simulink model "P642_VTS_Reference"  (R2026b)
settings: Solver=FixedStepDiscrete  StopTime=5  FixedStep=0.001
libraries: simulink_extras x4
settings Model: Creator=Medha Trust  LastModifiedBy=Medha Trust
settings DataIOCC: ExternalInput=input_data  LoadExternalInput=on

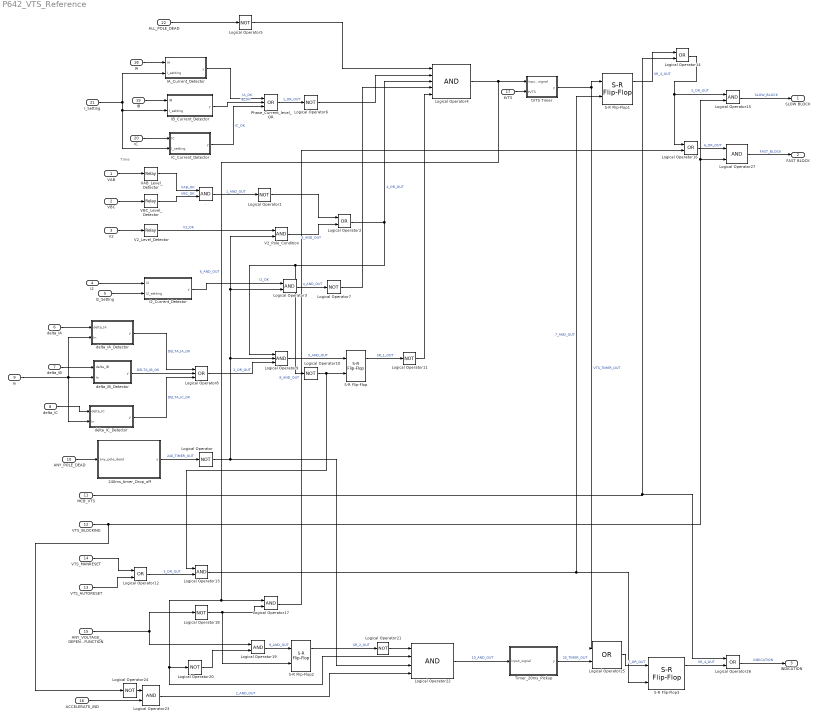
== system P642_VTS_Reference ==
  note: Time
  VAB : Inport
  VBC : Inport  Port=2
  V2 : Inport  Port=3  OutDataTypeStr=double
  I2 : Inport  Port=4
  I2_Setting : Inport  Port=5
  delta_IA : Inport  Port=6
  delta_IB : Inport  Port=7
  delta_IC : Inport  Port=8
  In : Inport  Port=9
  ANY_POLE_DEAD : Inport  Port=10
  MCB_VTS : Inport  Port=11  OutDataTypeStr=double
  VTS_BLOCKING : Inport  Port=12  OutDataTypeStr=double
  VTS_AUTORESET : Inport  Port=13  OutDataTypeStr=double
  VTS_MANRESET : Inport  Port=14  OutDataTypeStr=double
  ANY_VOLTAGE_DEPENDENT_FUNCTION : Inport  Port=15  OutDataTypeStr=double
  ACCELERATE_IND : Inport  Port=16  OutDataTypeStr=double
  tVTS : Inport  Port=17
  IA : Inport  Port=18
  IB : Inport  Port=19
  IC : Inport  Port=20
  I_Setting : Inport  Port=21
  ALL_POLE_DEAD : Inport  Port=22  OutDataTypeStr=double
  " ." : Logic  AllPortsSameDT=off  OutDataTypeStr=boolean
  240ms_timer_Drop_off : MATLAB Function  TreatAsAtomicUnit=on
  I2_Current_Detector : MATLAB Function  TreatAsAtomicUnit=on
  IA_Current_Detector : MATLAB Function  TreatAsAtomicUnit=on
  IB_Current_Detector : MATLAB Function  TreatAsAtomicUnit=on
  IC_Current_Detector : MATLAB Function  TreatAsAtomicUnit=on
  Logical Operator{,1,5..7,10..11,18,20..21,24} (11 alike) : Logic  Operator=NOT  AllPortsSameDT=off  OutDataTypeStr=boolean
  Logical Operator{2,12,14,16,25..26} (6 alike) : Logic  Operator=OR  AllPortsSameDT=off  OutDataTypeStr=boolean
  Logical Operator{3,13,15,17,19,23,27} (7 alike) : Logic  AllPortsSameDT=off  OutDataTypeStr=boolean
  Logical Operator22 : Logic  Inputs=4  AllPortsSameDT=off  OutDataTypeStr=boolean
  Logical Operator4 : Logic  Inputs=5  AllPortsSameDT=off  OutDataTypeStr=boolean
  Logical Operator8 : Logic  Operator=OR  Inputs=3  AllPortsSameDT=off  OutDataTypeStr=boolean
  Logical Operator9 : Logic  Inputs=3  AllPortsSameDT=off  OutDataTypeStr=boolean
  Phase_Current_level_OR : Logic  Operator=OR  Inputs=3  AllPortsSameDT=off  OutDataTypeStr=boolean
  S-R Flip-Flop{,1..3} (4 alike) : simulink_extras/Flip Flops/S-R Flip-Flop  initial_condition=0
  Timer_20ms_Pickup : MATLAB Function  TreatAsAtomicUnit=on
  V2_Level_Detector : Relay  OnSwitchValue=10  OffSwitchValue=9.5
  V2_Pole_Condition : Logic  AllPortsSameDT=off  OutDataTypeStr=boolean
  VAB_Level_Detector : Relay  OnSwitchValue=95  OffSwitchValue=70
  VBC_Level_Detector : Relay  OnSwitchValue=95  OffSwitchValue=70
  delta_IA_Detector : MATLAB Function  TreatAsAtomicUnit=on
  delta_IB_Detector : MATLAB Function  TreatAsAtomicUnit=on
  delta_IC_Detector : MATLAB Function  TreatAsAtomicUnit=on
  tVTS Timer : MATLAB Function  TreatAsAtomicUnit=on
  SLOW BLOCK : Outport
  FAST BLOCK : Outport  Port=2
  INDICATION : Outport  Port=3
  wires:
  VAB/1 -> VAB_Level_Detector/1
  VAB_Level_Detector/1 -> " ."/1  "VAB_OK"
  VBC/1 -> VBC_Level_Detector/1
  VBC_Level_Detector/1 -> " ."/2  "VBC_OK"
  V2/1 -> V2_Level_Detector/1
  V2_Level_Detector/1 -> V2_Pole_Condition/1  "V2_OK"
  I2/1 -> I2_Current_Detector/1(I2)
  I2_Setting/1 -> I2_Current_Detector/2(I2_setting)
  I2_Current_Detector/1(y) -> Logical Operator3/1  "I2_OK"
  delta_IA/1 -> delta_IA_Detector/1(delta_IA)
  In/1 -> delta_IC_Detector/2(In), delta_IB_Detector/2(In), delta_IA_Detector/2(In)
  delta_IB/1 -> delta_IB_Detector/1(delta_IB)
  delta_IC/1 -> delta_IC_Detector/1(delta_IC)
  Logical Operator/1 -> Logical Operator22/3, Logical Operator3/2, V2_Pole_Condition/2, Logical Operator9/2
  " ."/1 -> Logical Operator1/1  "1_AND_OUT"
  Logical Operator1/1 -> Logical Operator2/1
  V2_Pole_Condition/1 -> Logical Operator2/2  "3_AND_OUT"
  IB_Current_Detector/1(y) -> Phase_Current_level_OR/2  "IB_OK"
  IC/1 -> IC_Current_Detector/1(IC)
  IB/1 -> IB_Current_Detector/1(IB)
  I_Setting/1 -> IA_Current_Detector/2(I_setting), IC_Current_Detector/2(I_setting), IB_Current_Detector/2(I_setting)
  IA/1 -> IA_Current_Detector/1(IA)
  IC_Current_Detector/1(y) -> Phase_Current_level_OR/3  "IC_OK"
  IA_Current_Detector/1(y) -> Phase_Current_level_OR/1  "IA_OK"
  ALL_POLE_DEAD/1 -> Logical Operator5/1
  Logical Operator5/1 -> Logical Operator4/1
  Phase_Current_level_OR/1 -> Logical Operator6/1  "1_OR_OUT"
  Logical Operator6/1 -> Logical Operator4/2
  Logical Operator2/1 -> Logical Operator10/1, Logical Operator9/1, Logical Operator4/3  "4_OR_OUT"
  Logical Operator3/1 -> Logical Operator7/1  "4_AND_OUT"
  Logical Operator7/1 -> Logical Operator4/4
  delta_IA_Detector/1(y) -> Logical Operator8/1  "DELTA_IA_OK"
  delta_IB_Detector/1(y) -> Logical Operator8/2  "DELTA_IB_OK"
  delta_IC_Detector/1(y) -> Logical Operator8/3  "DELTA_IC_OK"
  Logical Operator8/1 -> Logical Operator9/3  "2_OR_OUT"
  Logical Operator9/1 -> S-R Flip-Flop/1  "5_AND_OUT"
  Logical Operator10/1 -> Logical Operator13/1, S-R Flip-Flop/2
  S-R Flip-Flop/1 -> Logical Operator11/1  "SR_1_OUT"
  Logical Operator11/1 -> Logical Operator4/5
  VTS_MANRESET/1 -> Logical Operator12/1
  VTS_AUTORESET/1 -> Logical Operator12/2
  Logical Operator12/1 -> Logical Operator13/2  "3_OR_OUT"
  tVTS/1 -> tVTS Timer/2(tVTS)
  Logical Operator4/1 -> tVTS Timer/1(input_signal), Logical Operator17/1, Logical Operator22/2, Logical Operator20/1  "6_AND_OUT"
  Logical Operator13/1 -> S-R Flip-Flop3/2, S-R Flip-Flop1/2  "7_AND_OUT"
  S-R Flip-Flop1/1 -> Logical Operator14/1  "SR_3_OUT"
  MCB_VTS/1 -> Logical Operator26/1, Logical Operator14/2
  Logical Operator14/1 -> Logical Operator15/1, Logical Operator16/1  "5_OR_OUT"
  VTS_BLOCKING/1 -> Logical Operator27/2, Logical Operator15/2, Logical Operator24/1
  ANY_VOLTAGE_DEPENDENT_FUNCTION/1 -> Logical Operator19/1, Logical Operator18/1
  Logical Operator18/1 -> S-R Flip-Flop2/2, Logical Operator17/2
  Logical Operator17/1 -> Logical Operator16/2  "8_AND_OUT"
  Logical Operator20/1 -> Logical Operator19/2
  Logical Operator19/1 -> S-R Flip-Flop2/1  "9_AND_OUT"
  S-R Flip-Flop2/1 -> Logical Operator21/1  "SR_2_OUT"
  Logical Operator21/1 -> Logical Operator22/1
  Logical Operator24/1 -> Logical Operator23/1
  ACCELERATE_IND/1 -> Logical Operator23/2
  Logical Operator23/1 -> Logical Operator22/4  "2_AND_OUT"
  ANY_POLE_DEAD/1 -> 240ms_timer_Drop_off/1(any_pole_dead)
  240ms_timer_Drop_off/1(y) -> Logical Operator/1  "240_TIMER_OUT"
  tVTS Timer/1(y) -> S-R Flip-Flop1/1, Logical Operator25/1  "VTS_TIMER_OUT"
  Logical Operator22/1 -> Timer_20ms_Pickup/1(input_signal)  "10_AND_OUT"
  Timer_20ms_Pickup/1(y) -> Logical Operator25/2  "20_TIMER_OUT"
  Logical Operator25/1 -> S-R Flip-Flop3/1  "7_OR_OUT"
  S-R Flip-Flop3/1 -> Logical Operator26/2  "SR_4_OUT"
  Logical Operator16/1 -> Logical Operator27/1  "6_OR_OUT"
  Logical Operator26/1 -> INDICATION/1  "INDICATION"
  Logical Operator27/1 -> FAST BLOCK/1  "FAST_BLOCK"
  Logical Operator15/1 -> SLOW BLOCK/1  "SLOW_BLOCK"

== matlab function P642_VTS_Reference/IA_Current_Detector ==
  data: IA input; y output; I_setting input
function y = fcn(IA, I_setting)
% P642 IA> current level detector
% Pickup  = 100% of I> setting
% Dropout = 95% of I> setting

persistent state

if isempty(state)
    state = 0;
end

pickup = I_setting;
dropout = 0.95 * I_setting;

if state == 0
    if abs(IA) >= pickup
        state = 1;
    end
else
    if abs(IA) < dropout
        state = 0;
    end
end

y = logical(state);

== matlab function P642_VTS_Reference/IC_Current_Detector ==
  data: IC input; y output; I_setting input
function y = fcn(IC, I_setting)

y=false; %Initializing input
% P642 IA> current level detector
% Pickup  = 100% of I> setting
% Dropout = 95% of I> setting

persistent state

if isempty(state)
    state = 0;
end

pickup = I_setting;
dropout = 0.95 * I_setting;

if state == 0
    if abs(IC) >= pickup
        state = 1;
    end
else
    if abs(IC) < dropout
        state = 0;
    end
end

y = logical(state);

== matlab function P642_VTS_Reference/I2_Current_Detector ==
  data: I2 input; y output boolean; I2_setting input
function y = fcn(I2, I2_setting)
% P642 I2> negative-sequence current detector
% Pickup  = 100% of I2> setting
% Dropout = 95% of I2> setting

persistent state

if isempty(state)
    state = 0;
end

pickup = I2_setting;
dropout = 0.95 * I2_setting;

if state == 0
    if abs(I2) >= pickup
        state = 1;
    end
else
    if abs(I2) < dropout
        state = 0;
    end
end

y = logical(state);

== matlab function P642_VTS_Reference/delta_IA_Detector ==
  data: delta_IA input; y output; In input
function y = fcn(delta_IA, In)
% P642 Delta IA> superimposed-current detector
% Threshold = 0.1 * In
% Operate decision must persist for 0.5 cycle
% Simulation step = 0.001 s
% Nominal frequency = 50 Hz
% Therefore 0.5 cycle = 0.01 s = 10 samples

persistent count state

if isempty(count)
    count = 0;
    state = 0;
end

threshold = 0.1 * In;
required_samples = 10;

if abs(delta_IA) >= threshold
    count = count + 1;
else
    count = 0;
    state = 0;
end

if count >= required_samples
    state = 1;
end

y = state;

== matlab function P642_VTS_Reference/delta_IB_Detector ==
  data: delta_IB input; y output; In input
function y = fcn(delta_IB, In)
% P642 Delta IA> superimposed-current detector
% Threshold = 0.1 * In
% Operate decision must persist for 0.5 cycle
% Simulation step = 0.001 s
% Nominal frequency = 50 Hz
% Therefore 0.5 cycle = 0.01 s = 10 samples

persistent count state

if isempty(count)
    count = 0;
    state = 0;
end

threshold = 0.1 * In;
required_samples = 10;

if abs(delta_IB) >= threshold
    count = count + 1;
else
    count = 0;
    state = 0;
end

if count >= required_samples
    state = 1;
end

y = state;

== matlab function P642_VTS_Reference/delta_IC_Detector ==
  data: delta_IC input; y output; In input
function y = fcn(delta_IC, In)

y=false; %Initializing input
% P642 Delta IA> superimposed-current detector
% Threshold = 0.1 * In
% Operate decision must persist for 0.5 cycle
% Simulation step = 0.001 s
% Nominal frequency = 50 Hz
% Therefore 0.5 cycle = 0.01 s = 10 samples

persistent count state

if isempty(count)
    count = 0;
    state = 0;
end

threshold = 0.1 * In;
required_samples = 10;

if abs(delta_IC) >= threshold
    count = count + 1;
else
    count = 0;
    state = 0;
end

if count >= required_samples
    state = 1;
end

y = state;

== matlab function P642_VTS_Reference/240ms_timer_Drop_off ==
  data: any_pole_dead input; y output
function y = fcn(any_pole_dead)

persistent state
persistent off_count

if isempty(state)
    state = 0;
    off_count = 0;
end

% 240 ms = 240 samples because Ts = 0.001 s
required_samples = 240;

if any_pole_dead == 1

    % Pickup is immediate
    state = 1;
    off_count = 0;

else

    % Drop-off is delayed
    if state == 1
        off_count = off_count + 1;

        if off_count >= required_samples
            state = 0;
            off_count = 0;
        end
    end

end

y = logical(state);

== matlab function P642_VTS_Reference/tVTS Timer ==
  data: input_signal input; y output; tVTS input

function y = fcn(input_signal, tVTS)
% Delayed pickup timer
% Assumes input_signal is Boolean and tVTS is in seconds.

persistent elapsed

if isempty(elapsed)
    elapsed = 0;
end

Ts = 0.001;  % Model sample time: 1 ms

if input_signal
    elapsed = elapsed + Ts;
else
    elapsed = 0;
end

y = input_signal && (elapsed >= tVTS);
end

== matlab function P642_VTS_Reference/Timer_20ms_Pickup ==
  data: input_signal input; y output
function y = fcn(input_signal)

persistent state
persistent on_count

if isempty(state)
    state = 0;
    on_count = 0;
end

% 20 ms = 20 samples because Ts = 0.001 s
required_samples = 20;

if input_signal == 1

    % Pickup is delayed
    on_count = on_count + 1;

    if on_count >= required_samples
        state = 1;
        on_count = 0;
    end

else

    % Drop-off is immediate
    state = 0;
    on_count = 0;

end

y = logical(state);

== matlab function P642_VTS_Reference/IB_Current_Detector ==
  data: IB input; y output; I_setting input
function y = fcn(IB, I_setting)
% P642 IA> current level detector
% Pickup  = 100% of I> setting
% Dropout = 95% of I> setting

persistent state

if isempty(state)
    state = 0;
end

pickup = I_setting;
dropout = 0.95 * I_setting;

if state == 0
    if abs(IB) >= pickup
        state = 1;
    end
else
    if abs(IB) < dropout
        state = 0;
    end
end

y = logical(state);
